simulink model "SatelliteTelescope_Architecture"  (R2023a)
settings: Solver=VariableStepAuto  StartTime=0.0  StopTime=300  RelTol=1e-3
settings Model: DataDictionary=SatelliteTelescope.sldd  Creator=Ren4  LastModifiedBy=Ren4
settings ModelReferenceCC: ModelReferenceMinAlgLoopOccurrences=on

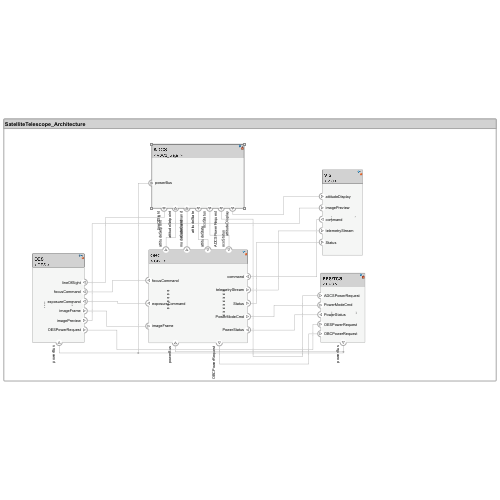
[thumbnail: Simulink's stored preview of the top-level diagram]
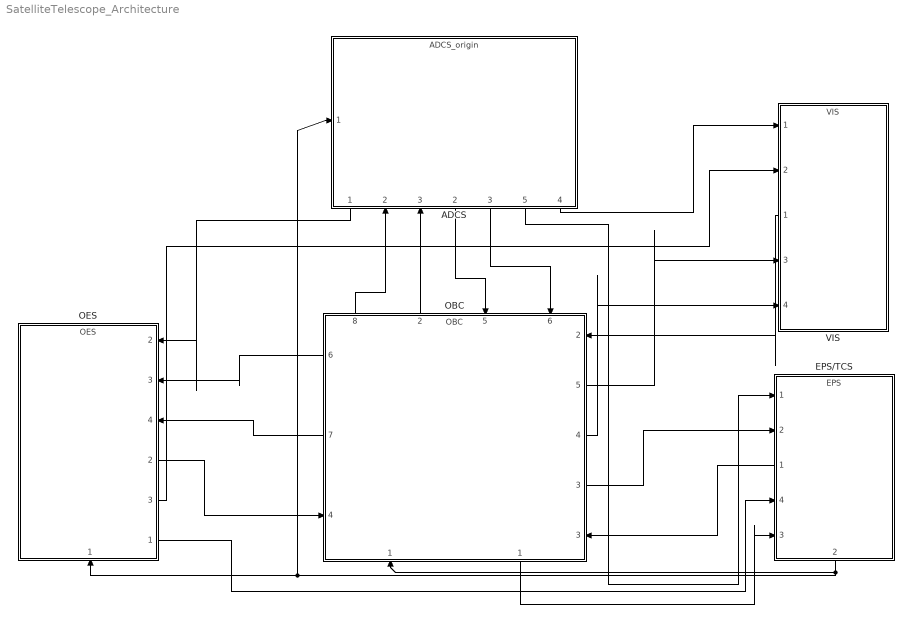
== system SatelliteTelescope_Architecture ==
  ADCS : ModelReference  ModelNameDialog=ADCS_origin  SimulationMode=Normal  ModelReferenceVersion=1.10
      settings: PortSchema="{\"entries\":[{\"content\":{\"headerSize\":38,\"margin\":15,\"minimumSpacing\":25,\"sides\":[{\"content\":{\"connectorIds\":[\"In1\"]},\"type\":\"ConnectorPlacement.EquallySpacedRectSide\",\"uuid\":\"ef56698f-e6b0-454c-8223-8f2ecac129c7\"},{\"content\":{\"side\":\"RIGHT\"},\"type\":\"ConnectorPlacement.EquallySpacedRectSide\",\"uuid\":\"db3ef4e7-07cc-43d4-a5b0-2ea8b0f7e660\"},{\"content\":{\"side\":\"TOP\"},\"type\":\"ConnectorPlacement.EquallySpacedRectSide\",\"uuid\":\"fa1a882f-6e8a-4b29-9591-ef9fd7276576\"},{\"content\":{\"connectorIds\":[\"Out1\",\"In2\",\"In3\",\"Out2\",\"Out3\",\"Out5\",\"Out4\"],\"side\":\"BOTTOM\"},\"type\":\"ConnectorPlacement.EquallySpacedRectSide\",\"uuid\":\"3a50c9ab-b5fe-483d-aae1-9c57e78d2e21\"}]},\"type\":\"ConnectorPlacement.EquallySpacedConnector\",\"uuid\":\"85df4891-9028-42bb-b4b6-79c96e1241b8\"}],\"packageUris\":[\"http://schema.mathworks.com/mf0/Connector/R2020b\"],\"version\":\"1.0\"}"
  EPS/TCS : ModelReference  ModelNameDialog=EPS  SimulationMode=Normal  ModelReferenceVersion=1.1
      settings: PortSchema="{\"entries\":[{\"content\":{\"headerSize\":38,\"margin\":15,\"minimumSpacing\":25,\"sides\":[{\"content\":{\"connectorIds\":[\"In1\",\"In2\",\"Out1\",\"In4\",\"In3\"]},\"type\":\"ConnectorPlacement.EquallySpacedRectSide\",\"uuid\":\"ef56698f-e6b0-454c-8223-8f2ecac129c7\"},{\"content\":{\"side\":\"RIGHT\"},\"type\":\"ConnectorPlacement.EquallySpacedRectSide\",\"uuid\":\"db3ef4e7-07cc-43d4-a5b0-2ea8b0f7e660\"},{\"content\":{\"side\":\"TOP\"},\"type\":\"ConnectorPlacement.EquallySpacedRectSide\",\"uuid\":\"fa1a882f-6e8a-4b29-9591-ef9fd7276576\"},{\"content\":{\"connectorIds\":[\"Out2\"],\"side\":\"BOTTOM\"},\"type\":\"ConnectorPlacement.EquallySpacedRectSide\",\"uuid\":\"72da216a-a726-4fe0-9092-f1edf9ed4d00\"}]},\"type\":\"ConnectorPlacement.EquallySpacedConnector\",\"uuid\":\"85df4891-9028-42bb-b4b6-79c96e1241b8\"}],\"packageUris\":[\"http://schema.mathworks.com/mf0/Connector/R2020b\"],\"version\":\"1.0\"}"
  OBC : ModelReference  ModelNameDialog=OBC  SimulationMode=Normal  ModelReferenceVersion=1.10
      settings: PortSchema="{\"entries\":[{\"content\":{\"headerSize\":38,\"margin\":15,\"minimumSpacing\":25,\"sides\":[{\"content\":{\"connectorIds\":[\"Out6\",\"Out7\",\"In4\"]},\"type\":\"ConnectorPlacement.EquallySpacedRectSide\",\"uuid\":\"ef56698f-e6b0-454c-8223-8f2ecac129c7\"},{\"content\":{\"connectorIds\":[\"In2\",\"Out5\",\"Out4\",\"Out3\",\"In3\"],\"side\":\"RIGHT\"},\"type\":\"ConnectorPlacement.EquallySpacedRectSide\",\"uuid\":\"db3ef4e7-07cc-43d4-a5b0-2ea8b0f7e660\"},{\"content\":{\"connectorIds\":[\"Out8\",\"Out2\",\"In5\",\"In6\"],\"side\":\"TOP\"},\"type\":\"ConnectorPlacement.EquallySpacedRectSide\",\"uuid\":\"fa1a882f-6e8a-4b29-9591-ef9fd7276576\"},{\"content\":{\"connectorIds\":[\"In1\",\"Out1\"],\"side\":\"BOTTOM\"},\"type\":\"ConnectorPlacement.EquallySpacedRectSide\",\"uuid\":\"fe9a0636-c72d-4296-83f6-a16dd9ec1870\"}]},\"type\":\"ConnectorPlacement.EquallySpacedConnector\",\"uuid\":\"85df4891-9028-42bb-b4b6-79c96e1241b8\"}],\"packageUris\":[\"http://schema.mathworks.com/mf0/Connector/R2020b\"],\"version\":\"1.0\"}"
  OES : ModelReference  ModelNameDialog=OES  SimulationMode=Normal  ModelReferenceVersion=1.1
      settings: PortSchema="{\"entries\":[{\"content\":{\"headerSize\":38,\"margin\":15,\"minimumSpacing\":25,\"sides\":[{\"content\":{},\"type\":\"ConnectorPlacement.EquallySpacedRectSide\",\"uuid\":\"ef56698f-e6b0-454c-8223-8f2ecac129c7\"},{\"content\":{\"connectorIds\":[\"In2\",\"In3\",\"In4\",\"Out2\",\"Out3\",\"Out1\"],\"side\":\"RIGHT\"},\"type\":\"ConnectorPlacement.EquallySpacedRectSide\",\"uuid\":\"db3ef4e7-07cc-43d4-a5b0-2ea8b0f7e660\"},{\"content\":{\"side\":\"TOP\"},\"type\":\"ConnectorPlacement.EquallySpacedRectSide\",\"uuid\":\"fa1a882f-6e8a-4b29-9591-ef9fd7276576\"},{\"content\":{\"connectorIds\":[\"In1\"],\"side\":\"BOTTOM\"},\"type\":\"ConnectorPlacement.EquallySpacedRectSide\",\"uuid\":\"f7b65001-5802-429d-a250-6d52ab461aa7\"}]},\"type\":\"ConnectorPlacement.EquallySpacedConnector\",\"uuid\":\"85df4891-9028-42bb-b4b6-79c96e1241b8\"}],\"packageUris\":[\"http://schema.mathworks.com/mf0/Connector/R2020b\"],\"version\":\"1.0\"}"
  VIS : ModelReference  ModelNameDialog=VIS  SimulationMode=Normal  ModelReferenceVersion=1.1
      settings: PortSchema="{\"entries\":[{\"content\":{\"headerSize\":38,\"margin\":15,\"minimumSpacing\":25,\"sides\":[{\"content\":{\"connectorIds\":[\"In1\",\"In2\",\"Out1\",\"In3\",\"In4\"]},\"type\":\"ConnectorPlacement.EquallySpacedRectSide\",\"uuid\":\"ef56698f-e6b0-454c-8223-8f2ecac129c7\"},{\"content\":{\"side\":\"RIGHT\"},\"type\":\"ConnectorPlacement.EquallySpacedRectSide\",\"uuid\":\"db3ef4e7-07cc-43d4-a5b0-2ea8b0f7e660\"},{\"content\":{\"side\":\"TOP\"},\"type\":\"ConnectorPlacement.EquallySpacedRectSide\",\"uuid\":\"fa1a882f-6e8a-4b29-9591-ef9fd7276576\"},{\"content\":{\"side\":\"BOTTOM\"},\"type\":\"ConnectorPlacement.EquallySpacedRectSide\",\"uuid\":\"da977ad7-9925-4433-9c89-5bbb77277070\"}]},\"type\":\"ConnectorPlacement.EquallySpacedConnector\",\"uuid\":\"85df4891-9028-42bb-b4b6-79c96e1241b8\"}],\"packageUris\":[\"http://schema.mathworks.com/mf0/Connector/R2020b\"],\"version\":\"1.0\"}"
  wires:
  ADCS/2 -> OBC/5
  ADCS/3 -> OBC/6
  OBC/8 -> ADCS/2
  OBC/2 -> ADCS/3
  OBC/7 -> OES/4
  OBC/6 -> OES/3
  ADCS/1 -> OES/2
  OES/2 -> OBC/4
  OBC/4 -> VIS/4
  ADCS/4 -> VIS/1
  OES/3 -> VIS/2
  OBC/5 -> VIS/3
  VIS/1 -> OBC/2
  ADCS/5 -> EPS/TCS/1
  OBC/1 -> EPS/TCS/3
  OES/1 -> EPS/TCS/4
  OBC/3 -> EPS/TCS/2
  EPS/TCS/1 -> OBC/3
  EPS/TCS/2 -> ADCS/1, OES/1, OBC/1
